simulink model "ev_powertrain_gokart"  (R2025b)
settings: Solver=ode23tb  StartTime=0.0  StopTime=150  RelTol=1e-3
undefined symbols (not defined in the file or in its folder): DiscIntNeverNeededParam
libraries: simulink x3
settings Model: Creator=dhairyarajsinghshekhawat  LastModifiedBy=dhairyarajsinghshekhawat

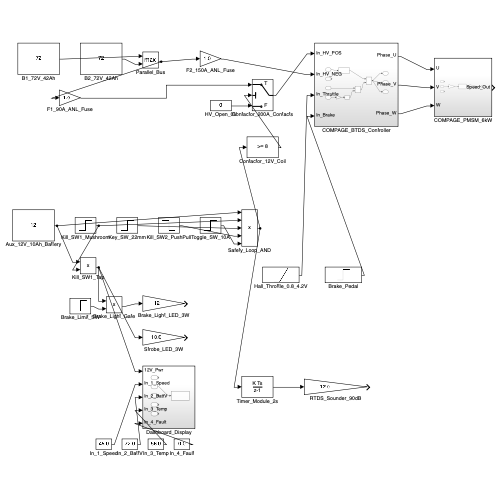
[thumbnail: Simulink's stored preview of the top-level diagram]
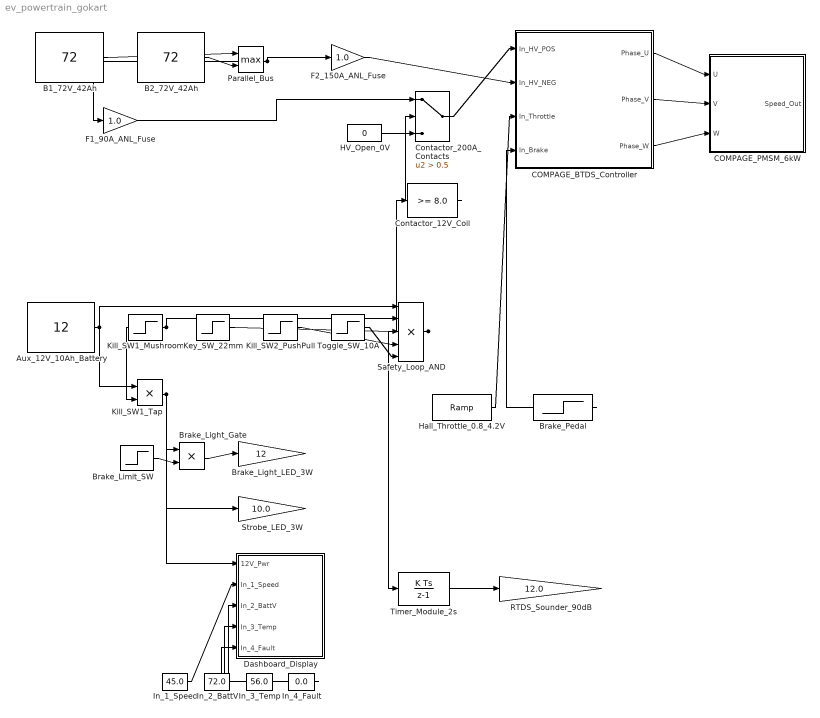
== system ev_powertrain_gokart ==
  Aux_12V_10Ah_Battery : Constant  Value=12
  B1_72V_42Ah : Constant  Value=72
  B2_72V_42Ah : Constant  Value=72
  Brake_Light_Gate : Product
  Brake_Light_LED_3W : Gain  Gain=12
  Brake_Limit_SW : Step  Time=1.2  SampleTime=0
  Brake_Pedal : Step  Time=3.2  SampleTime=0
  COMPAGE_BTDS_Controller : Subsystem
  COMPAGE_PMSM_6kW : Subsystem
  Contactor_12V_Coil : simulink/Logic and Bit Operations/Compare To Constant  relop=>=  const=8.0  OutDataTypeStr=boolean
  Contactor_200A_Contacts : Switch  Criteria=u2 > Threshold  Threshold=0.5  SaturateOnIntegerOverflow=off  InputSameDT=off
  Dashboard_Display : Subsystem
  F1_90A_ANL_Fuse : Gain  Gain=1.0
  F2_150A_ANL_Fuse : Gain  Gain=1.0
  HV_Open_0V : Constant  Value=0
  Hall_Throttle_0.8_4.2V : simulink/Sources/Ramp  slope=0.4  start=2.0  InitialOutput=0
  In_1_Speed : Constant  Value=45.0
  In_2_BattV : Constant  Value=72.0
  In_3_Temp : Constant  Value=56.0
  In_4_Fault : Constant  Value=0.0
  Key_SW_22mm : Step  Time=0.2  SampleTime=0
  Kill_SW1_Mushroom : Step  Time=0.1  SampleTime=0
  Kill_SW1_Tap : Product
  Kill_SW2_PushPull : Step  Time=4.5  Before=1  After=0  SampleTime=0
  Parallel_Bus : MinMax  Function=max  Inputs=2
  RTDS_Sounder_90dB : Gain  Gain=12.0
  Safety_Loop_AND : Product  Inputs=5
  Strobe_LED_3W : Gain  Gain=10.0
  Timer_Module_2s : DiscreteIntegrator  SampleTime=-1  ICPrevOutput=DiscIntNeverNeededParam  ICPrevScaledInput=DiscIntNeverNeededParam
  Toggle_SW_10A : Step  Time=0.5  SampleTime=0
  wires:
  B1_72V_42Ah/1 -> Parallel_Bus/1
  B2_72V_42Ah/1 -> Parallel_Bus/2
  Parallel_Bus/1 -> F1_90A_ANL_Fuse/1, F2_150A_ANL_Fuse/1
  Contactor_12V_Coil/1 -> Contactor_200A_Contacts/2
  HV_Open_0V/1 -> Contactor_200A_Contacts/3
  Contactor_200A_Contacts/1 -> COMPAGE_BTDS_Controller/1(In_HV_POS)
  F2_150A_ANL_Fuse/1 -> COMPAGE_BTDS_Controller/2(In_HV_NEG)
  COMPAGE_BTDS_Controller/1(Phase_U) -> COMPAGE_PMSM_6kW/1(U)
  COMPAGE_BTDS_Controller/2(Phase_V) -> COMPAGE_PMSM_6kW/2(V)
  COMPAGE_BTDS_Controller/3(Phase_W) -> COMPAGE_PMSM_6kW/3(W)
  Aux_12V_10Ah_Battery/1 -> Safety_Loop_AND/1, Kill_SW1_Tap/1
  Kill_SW1_Mushroom/1 -> Safety_Loop_AND/2, Kill_SW1_Tap/2
  Key_SW_22mm/1 -> Safety_Loop_AND/3
  Kill_SW2_PushPull/1 -> Safety_Loop_AND/4
  Toggle_SW_10A/1 -> Safety_Loop_AND/5
  Kill_SW1_Tap/1 -> Brake_Light_Gate/1, Strobe_LED_3W/1, Dashboard_Display/1(12V_Pwr)
  Brake_Limit_SW/1 -> Brake_Light_Gate/2
  Brake_Light_Gate/1 -> Brake_Light_LED_3W/1
  In_1_Speed/1 -> Dashboard_Display/2(In_1_Speed)
  In_2_BattV/1 -> Dashboard_Display/3(In_2_BattV)
  In_3_Temp/1 -> Dashboard_Display/4(In_3_Temp)
  In_4_Fault/1 -> Dashboard_Display/5(In_4_Fault)
  Safety_Loop_AND/1 -> Contactor_12V_Coil/1, Timer_Module_2s/1
  Timer_Module_2s/1 -> RTDS_Sounder_90dB/1
  Hall_Throttle_0.8_4.2V/1 -> COMPAGE_BTDS_Controller/3(In_Throttle)
  Brake_Pedal/1 -> COMPAGE_BTDS_Controller/4(In_Brake)
  F1_90A_ANL_Fuse/1 -> Contactor_200A_Contacts/1

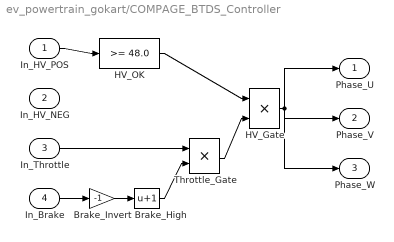
== system ev_powertrain_gokart/COMPAGE_BTDS_Controller ==
  In_HV_POS : Inport
  In_HV_NEG : Inport  Port=2
  In_Throttle : Inport  Port=3
  In_Brake : Inport  Port=4
  Brake_High : Bias  Bias=1  SaturateOnIntegerOverflow=off
  Brake_Invert : Gain  Gain=-1
  HV_Gate : Product
  HV_OK : simulink/Logic and Bit Operations/Compare To Constant  relop=>=  const=48.0  OutDataTypeStr=boolean
  Throttle_Gate : Product
  Phase_U : Outport
  Phase_V : Outport  Port=2
  Phase_W : Outport  Port=3
  wires:
  In_Brake/1 -> Brake_Invert/1
  Brake_Invert/1 -> Brake_High/1
  In_Throttle/1 -> Throttle_Gate/1
  Brake_High/1 -> Throttle_Gate/2
  In_HV_POS/1 -> HV_OK/1
  HV_OK/1 -> HV_Gate/1
  Throttle_Gate/1 -> HV_Gate/2
  HV_Gate/1 -> Phase_U/1, Phase_V/1, Phase_W/1

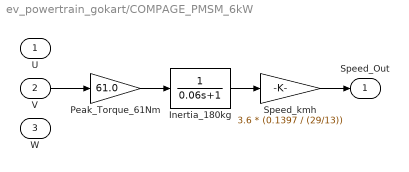
== system ev_powertrain_gokart/COMPAGE_PMSM_6kW ==
  U : Inport
  V : Inport  Port=2
  W : Inport  Port=3
  Inertia_180kg : TransferFcn  Denominator=[0.06 1]
  Peak_Torque_61Nm : Gain  Gain=61.0
  Speed_kmh : Gain  Gain=3.6 * (0.1397 / (29/13))
  Speed_Out : Outport
  wires:
  V/1 -> Peak_Torque_61Nm/1
  Peak_Torque_61Nm/1 -> Inertia_180kg/1
  Inertia_180kg/1 -> Speed_kmh/1
  Speed_kmh/1 -> Speed_Out/1

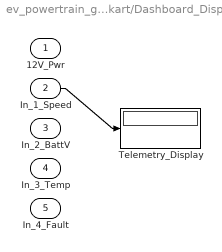
== system ev_powertrain_gokart/Dashboard_Display ==
  12V_Pwr : Inport
  In_1_Speed : Inport  Port=2
  In_2_BattV : Inport  Port=3
  In_3_Temp : Inport  Port=4
  In_4_Fault : Inport  Port=5
  Telemetry_Display : Display
  wires:
  In_1_Speed/1 -> Telemetry_Display/1
